simulink model "Lab3_2_3_1"  (R2024b)
settings: Solver=VariableStepAuto  StartTime=0.0  StopTime=3  RelTol=1e-3
undefined symbols (not defined in the file): A, B, D, K, Nr
libraries: simulink_extras x2
settings Model: Creator=vahid  LastModifiedBy=vahid

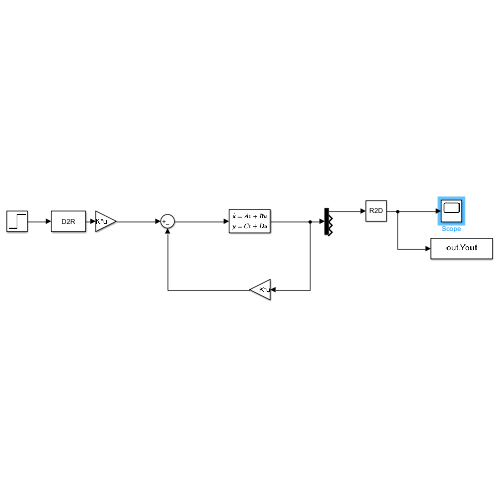
[thumbnail: Simulink's stored preview of the top-level diagram]
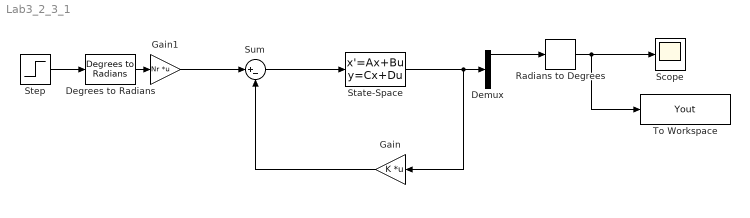
== system Lab3_2_3_1 ==
  Degrees to Radians : simulink_extras/Transformations/Degrees to Radians
  Demux : Demux
  Gain : Gain  Gain=K  Multiplication=Matrix(K*u)
  Gain1 : Gain  Gain=Nr  Multiplication=Matrix(K*u)
  Radians to Degrees : simulink_extras/Transformations/Radians to Degrees
  Scope : Scope
  State-Space : StateSpace  A=A  B=B  C=eye(4)  D=D  InitialCondition=0
  Step : Step  Time=0  After=50  SampleTime=0
  Sum : Sum  Inputs=|+-
  To Workspace : ToWorkspace  VariableName=Yout  SaveFormat=Timeseries  SampleTime=-1
  wires:
  State-Space/1 -> Demux/1, Gain/1
  Step/1 -> Degrees to Radians/1
  Sum/1 -> State-Space/1
  Gain/1 -> Sum/2
  Gain1/1 -> Sum/1
  Demux/1 -> Radians to Degrees/1
  Degrees to Radians/1 -> Gain1/1
  Radians to Degrees/1 -> To Workspace/1, Scope/1
